simulink model "PowerSplitHEV_system_model"  (R2023a)
settings: Solver=daessc  StartTime=0.0  StopTime=t_end  RelTol=1e-3  AbsTol=1e-3  EnableMultiTasking=on
PreLoadFcn:
  | PowerSplitHEV_params
  | 
  | PowerSplitHEV_DirectInput_selectInput
PostLoadFcn:
  | % Load external input signals
  | % based on the referenced subsystem
  | % for the Controller & Environment block.
  | PowerSplitHEV_system_model_setup
libraries: fl_lib x1, nesl_utility x1
settings Model: Creator=MathWorks  LastModifiedBy=isaacito
settings SolverCC: AutoScaleAbsTol=off  DaesscMode=Fast  AlgebraicLoopSolver=TrustRegion
settings DataIOCC: LimitDataPoints=on  MaxDataPoints=15000  SaveFormat=Array  DSMLogging=off  InspectSignalLogs=on
settings OptimizationCC: ReuseModelBlockBuffer=off  ExpressionDepthLimit=2147483647  LifeSpan=inf
settings DebuggingCC: UnconnectedInputMsg=warning  UnconnectedOutputMsg=warning  UnconnectedLineMsg=warning  StateNameClashWarn=warning  SFUnexpectedBacktrackingDiag=warning  SFNoUnconditionalDefaultTransitionDiag=warning  SFExecutionAtInitializationDiag=none  ArithmeticOperatorsInVariantConditions=warning
settings HardwareCC: ProdBitPerPointer=32  ProdBitPerSizeT=32  ProdBitPerPtrDiffT=32  ProdLargestAtomicFloat=None  ProdIntDivRoundTo=Undefined  ProdEndianess=Unspecified  ProdWordSize=32  ProdHWDeviceType=32-bit Generic
settings ModelReferenceCC: EnableRefExpFcnMdlSchedulingChecks=on  PropagateSignalLabelsOutOfModel=off
settings SFSimCC: SimUseLocalCustomCode=off  CustomCodeUndefinedFunction=UseInterfaceOnly
settings RTWCC: RTWUseLocalCustomCode=off  DLArmComputeVersion=19.05
settings CodeAppCC: StateflowObjectComments=on
settings GRTTargetCC: TargetLangStandard=C89/C90 (ANSI)  CombineOutputUpdateFcns=off  GRTInterface=on
settings ConfigComp: CovMetricSettings=dw  CovSaveCumulativeToWorkspaceVar=on  CovSaveSingleToWorkspaceVar=on  CovExternalEMLEnable=off
settings SimscapeCC: SimscapeLogType=all  SimscapeLogSimulationStatistics=on  SimscapeLogLimitData=off  SimscapeLogDataHistory=10000

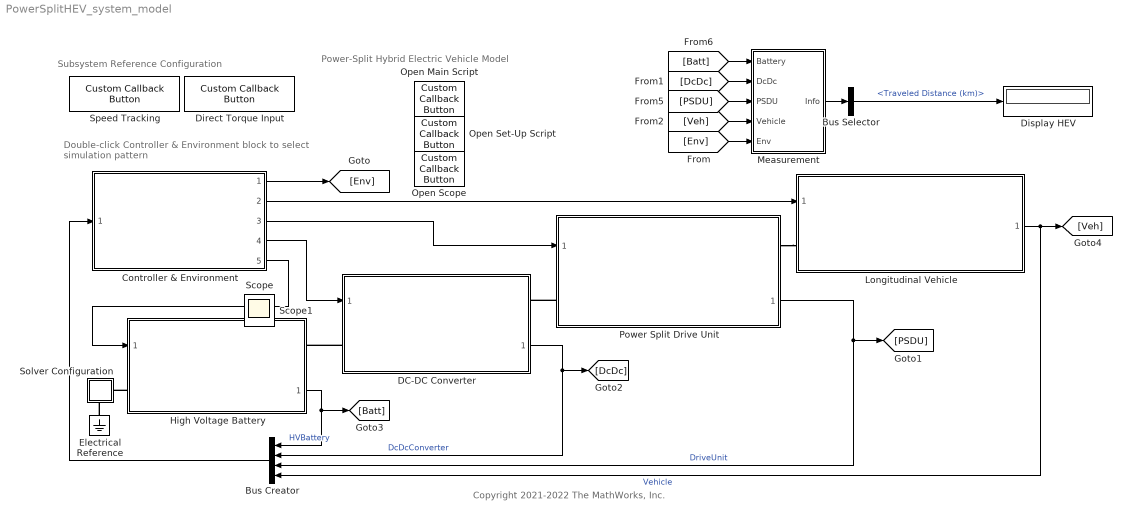
== system PowerSplitHEV_system_model ==
  note: Double-click Controller & Environment block
      | to select simulation pattern
  note: Subsystem Reference Configuration
  note: Power-Split Hybrid Electric Vehicle Model
  note: Copyright 2021-2022 The MathWorks, Inc.
  Bus Creator : BusCreator  Inputs=4
  Bus Selector : BusSelector  OutputSignals=Traveled Distance (km)
  Controller & Environment : Subsystem  ReferencedSubsystem=PowerSplitHEV_SpeedTracking_refsub
  DC-DC Converter : Subsystem  ReferencedSubsystem=DcDcConverterElec_refsub
      settings: PortSchema="{\"entries\":[{\"content\":{\"sides\":[{\"content\":{\"connectorIds\":[\"In1\",\"LConn1\"]},\"type\":\"ConnectorPlacement.EquallySpacedRectSide\",\"uuid\":\"9fe8411b-04be-463e-9924-e5b159c802ea\"},{\"content\":{\"connectorIds\":[\"RConn1\",\"Out1\"],\"side\":\"RIGHT\"},\"type\":\"ConnectorPlacement.EquallySpacedRectSide\",\"uuid\":\"f74ab51b-f871-4eba-ad48-2355a260a50e\"},{\"content\":{\"side\":\"TOP\"},\"type\":\"ConnectorPlacement.EquallySpacedRectSide\",\"uuid\":\"5fe4b190-e251-4a98-9e87-336539b68eba\"},{\"content\":{\"side\":\"HIDDEN\"},\"type\":\"ConnectorPlacement.EquallySpacedRectSide\",\"uuid\":\"70e61028-3020-42d1-b1c6-53691d04cdd7\"}]},\"type\":\"ConnectorPlacement.EquallySpacedConnector\",\"uuid\":\"64b2eeb8-79e5-4be4-98bc-81a0cbd61baa\"}],\"packageUris\":[\"http://schema.mathworks.com/mf0/Connector/R2020b\"],\"version\":\"1.0\"}"
  Direct Torque Input : CustomCallbackButton  Configuration="{\"components\":[{\"name\":\"BackgroundImageComponent\",\"settings\":{\"image\":{\"size\":[0,0],\"src\":\"default\",\"srcOrientation\":\"Right\"},\"position\":[0,0,1,1]}},{\"name\":\"ButtonStateComponent\",\"settings\":{\"buttonType\":\"momentary\",\"clickFcn\":\"disp(\\\"Selecting referenced subsystem: \\\" + ...\\n  \\\"Direct torque input\\\")\\n\\nset_param( gcs + \\\"\\/Controller & Environment\\\", ...\\n  \\\"ReferencedSubsystem\\\", ...\\n  \\\"PowerSplitHEV_DirectInput_refsub\\\");\\n\\nPowerSplitHEV_DirectInput_selectInput( ...\\n  \\\"InputPattern\\\", \\\"PowerSplitDrive\\\", ...\\n  \\\"DisplayMessage\\\", true );\\n\",\"onValue\":1,\"position\":[0,0,1,1],\"pressDelay\":\"500\",\"pressFcn\":\"\",\"repeatInterval\":\"0\",\"states\":[{\"horizontalAlignment\":\"center\",\"image\":{\"position\":[0,0,1,1],\"src\":\"default\",\"srcOrientation\":\"Right\"},\"label\":{\"color\":[0.01176470588,0.01176470588,0.01176470588,1],\"icon\":{\"size\":[0,0],\"src\":\"default\",\"srcOrientation\":\"Right\"},\"iconPlacement\":\"left\",\"text\":{\"content\":\"Select\"}},\"labelOffset\":[0,0],\"verticalAlignment\":\"middle\"},{\"horizontalAlignment\":\"center\",\"image\":{\"position\":[0,0,1,1],\"src\":\"default\",\"srcOrientation\":\"Right\"},\"label\":{\"color\":[0.01176470588,0.01176470588,0.01176470588,1],\"icon\":{\"size\":[0,0],\"src\":\"default\",\"srcOrientation\":\"Right\"},\"iconPlacement\":\"left\",\"text\":{\"content\":\"Select\"}},\"labelOffset\":[0,0],\"verticalAlignment\":\"middle\"},{\"horizontalAlignment\":\"center\",\"image\":{\"position\":[0,0,1,1],\"src\":\"default\",\"srcOrientation\":\"Right\"},\"label\":{\"color\":[0.01176470588,0.01176470588,0.01176470588,1],\"icon\":{\"size\":[0,0],\"src\":\"default\",\"srcOrientation\":\"Right\"},\"iconPlacement\":\"left\",\"text\":{\"content\":\"Select\"}},\"labelOffset\":[0,0],\"verticalAlignment\":\"middle\"},{\"horizontalAlignment\":\"center\",\"image\":{\"position\":[0,0,1,1],\"src\":\"default\",\"srcOrientation\":\"Right\"},\"label\":{\"color\":[0.01176470588,0.01176470588,0.01176470588,1],\"icon\":{\"size\":[0,0],\"src\":\"default\",\"srcOrientation\":\"Right\"},\"iconPlacement\":\"left\",\"text\":{\"content\":\"Select\"}},\"labelOffset\":[0,0],\"verticalAlignment\":\"middle\"}]}},{\"name\":\"ForegroundImageComponent\",\"settings\":{\"image\":{\"size\":[0,0],\"src\":\"default\",\"srcOrientation\":\"Right\"},\"isForeground\":1,\"position\":[0,0,1,1]}}],\"settings\":{\"BindingType\":\"standalone\",\"backgroundColor\":[244,244,244,1],\"backgroundOffset\":0.2,\"backgroundOpacity\":1,\"fixedAspectRatio\":\"off\",\"foregroundColor\":[0.01176470588,0.01176470588,0.01176470588,1],\"migratedFromLegacy\":true,\"useBackgroundColor\":true,\"variant\":\"callback\",\"version\":\"R2023a\"},\"type\":\"Button\"}"  CustomBackgroundColor="{\"color\":[0.9568627451,0.9568627451,0.9568627451],\"show\":true}"
  Display HEV : Display
  Electrical Reference : fl_lib/Electrical/Electrical Elements/Electrical Reference
  High Voltage Battery : Subsystem  ReferencedSubsystem=BatteryHV_refsub_Basic
      settings: OpenFcn="open_system(gcb, \"force\")"  PortSchema="{\"entries\":[{\"content\":{\"sides\":[{\"content\":{\"connectorIds\":[\"In1\",\"LConn1\"]},\"type\":\"ConnectorPlacement.EquallySpacedRectSide\",\"uuid\":\"9fe8411b-04be-463e-9924-e5b159c802ea\"},{\"content\":{\"connectorIds\":[\"RConn1\",\"Out1\"],\"side\":\"RIGHT\"},\"type\":\"ConnectorPlacement.EquallySpacedRectSide\",\"uuid\":\"f74ab51b-f871-4eba-ad48-2355a260a50e\"},{\"content\":{\"side\":\"TOP\"},\"type\":\"ConnectorPlacement.EquallySpacedRectSide\",\"uuid\":\"5fe4b190-e251-4a98-9e87-336539b68eba\"},{\"content\":{\"side\":\"HIDDEN\"},\"type\":\"ConnectorPlacement.EquallySpacedRectSide\",\"uuid\":\"70e61028-3020-42d1-b1c6-53691d04cdd7\"}]},\"type\":\"ConnectorPlacement.EquallySpacedConnector\",\"uuid\":\"64b2eeb8-79e5-4be4-98bc-81a0cbd61baa\"}],\"packageUris\":[\"http://schema.mathworks.com/mf0/Connector/R2020b\"],\"version\":\"1.0\"}"
  Longitudinal Vehicle : Subsystem  ReferencedSubsystem=Vehicle1D_refsub_Basic
  Measurement : Subsystem
  Open Main Script : CustomCallbackButton  Configuration="{\"components\":[{\"name\":\"BackgroundImageComponent\",\"settings\":{\"image\":{\"size\":[0,0],\"src\":\"default\",\"srcOrientation\":\"Right\"},\"position\":[0,0,1,1]}},{\"name\":\"ButtonStateComponent\",\"settings\":{\"buttonType\":\"momentary\",\"clickFcn\":\"edit(\\\"PowerSplitHEV_main_script\\\")\\n\",\"onValue\":1,\"position\":[0,0,1,1],\"pressDelay\":\"500\",\"pressFcn\":\"\",\"repeatInterval\":\"0\",\"states\":[{\"horizontalAlignment\":\"center\",\"image\":{\"position\":[0,0,1,1],\"src\":\"default\",\"srcOrientation\":\"Right\"},\"label\":{\"color\":[0.01176470588,0.01176470588,0.01176470588,1],\"icon\":{\"size\":[0,0],\"src\":\"default\",\"srcOrientation\":\"Right\"},\"iconPlacement\":\"left\",\"text\":{\"content\":\"Open\"}},\"labelOffset\":[0,0],\"verticalAlignment\":\"middle\"},{\"horizontalAlignment\":\"center\",\"image\":{\"position\":[0,0,1,1],\"src\":\"default\",\"srcOrientation\":\"Right\"},\"label\":{\"color\":[0.01176470588,0.01176470588,0.01176470588,1],\"icon\":{\"size\":[0,0],\"src\":\"default\",\"srcOrientation\":\"Right\"},\"iconPlacement\":\"left\",\"text\":{\"content\":\"Open\"}},\"labelOffset\":[0,0],\"verticalAlignment\":\"middle\"},{\"horizontalAlignment\":\"center\",\"image\":{\"position\":[0,0,1,1],\"src\":\"default\",\"srcOrientation\":\"Right\"},\"label\":{\"color\":[0.01176470588,0.01176470588,0.01176470588,1],\"icon\":{\"size\":[0,0],\"src\":\"default\",\"srcOrientation\":\"Right\"},\"iconPlacement\":\"left\",\"text\":{\"content\":\"Open\"}},\"labelOffset\":[0,0],\"verticalAlignment\":\"middle\"},{\"horizontalAlignment\":\"center\",\"image\":{\"position\":[0,0,1,1],\"src\":\"default\",\"srcOrientation\":\"Right\"},\"label\":{\"color\":[0.01176470588,0.01176470588,0.01176470588,1],\"icon\":{\"size\":[0,0],\"src\":\"default\",\"srcOrientation\":\"Right\"},\"iconPlacement\":\"left\",\"text\":{\"content\":\"Open\"}},\"labelOffset\":[0,0],\"verticalAlignment\":\"middle\"}]}},{\"name\":\"ForegroundImageComponent\",\"settings\":{\"image\":{\"size\":[0,0],\"src\":\"default\",\"srcOrientation\":\"Right\"},\"isForeground\":1,\"position\":[0,0,1,1]}}],\"settings\":{\"BindingType\":\"standalone\",\"backgroundColor\":[244,244,244,1],\"backgroundOffset\":0.2,\"backgroundOpacity\":1,\"fixedAspectRatio\":\"off\",\"foregroundColor\":[0.01176470588,0.01176470588,0.01176470588,1],\"migratedFromLegacy\":true,\"useBackgroundColor\":true,\"variant\":\"callback\",\"version\":\"R2023a\"},\"type\":\"Button\"}"  CustomBackgroundColor="{\"color\":[0.9568627451,0.9568627451,0.9568627451],\"show\":true}"
  Open Scope : CustomCallbackButton  Configuration="{\"components\":[{\"name\":\"BackgroundImageComponent\",\"settings\":{\"image\":{\"size\":[0,0],\"src\":\"default\",\"srcOrientation\":\"Right\"},\"position\":[0,0,1,1]}},{\"name\":\"ButtonStateComponent\",\"settings\":{\"buttonType\":\"momentary\",\"clickFcn\":\"open_system(gcs + \\\"\\/Measurement\\/Scope HEV\\\")\",\"onValue\":1,\"position\":[0,0,1,1],\"pressDelay\":\"500\",\"pressFcn\":\"\",\"repeatInterval\":\"0\",\"states\":[{\"horizontalAlignment\":\"center\",\"image\":{\"position\":[0,0,1,1],\"src\":\"default\",\"srcOrientation\":\"Right\"},\"label\":{\"color\":[0.01176470588,0.01176470588,0.01176470588,1],\"icon\":{\"size\":[0,0],\"src\":\"default\",\"srcOrientation\":\"Right\"},\"iconPlacement\":\"left\",\"text\":{\"content\":\"Open\"}},\"labelOffset\":[0,0],\"verticalAlignment\":\"middle\"},{\"horizontalAlignment\":\"center\",\"image\":{\"position\":[0,0,1,1],\"src\":\"default\",\"srcOrientation\":\"Right\"},\"label\":{\"color\":[0.01176470588,0.01176470588,0.01176470588,1],\"icon\":{\"size\":[0,0],\"src\":\"default\",\"srcOrientation\":\"Right\"},\"iconPlacement\":\"left\",\"text\":{\"content\":\"Open\"}},\"labelOffset\":[0,0],\"verticalAlignment\":\"middle\"},{\"horizontalAlignment\":\"center\",\"image\":{\"position\":[0,0,1,1],\"src\":\"default\",\"srcOrientation\":\"Right\"},\"label\":{\"color\":[0.01176470588,0.01176470588,0.01176470588,1],\"icon\":{\"size\":[0,0],\"src\":\"default\",\"srcOrientation\":\"Right\"},\"iconPlacement\":\"left\",\"text\":{\"content\":\"Open\"}},\"labelOffset\":[0,0],\"verticalAlignment\":\"middle\"},{\"horizontalAlignment\":\"center\",\"image\":{\"position\":[0,0,1,1],\"src\":\"default\",\"srcOrientation\":\"Right\"},\"label\":{\"color\":[0.01176470588,0.01176470588,0.01176470588,1],\"icon\":{\"size\":[0,0],\"src\":\"default\",\"srcOrientation\":\"Right\"},\"iconPlacement\":\"left\",\"text\":{\"content\":\"Open\"}},\"labelOffset\":[0,0],\"verticalAlignment\":\"middle\"}]}},{\"name\":\"ForegroundImageComponent\",\"settings\":{\"image\":{\"size\":[0,0],\"src\":\"default\",\"srcOrientation\":\"Right\"},\"isForeground\":1,\"position\":[0,0,1,1]}}],\"settings\":{\"BindingType\":\"standalone\",\"backgroundColor\":[244,244,244,1],\"backgroundOffset\":0.2,\"backgroundOpacity\":1,\"fixedAspectRatio\":\"off\",\"foregroundColor\":[0.01176470588,0.01176470588,0.01176470588,1],\"migratedFromLegacy\":true,\"useBackgroundColor\":true,\"variant\":\"callback\",\"version\":\"R2023a\"},\"type\":\"Button\"}"  CustomBackgroundColor="{\"color\":[0.9568627451,0.9568627451,0.9568627451],\"show\":true}"
  Open Set-Up Script : CustomCallbackButton  Configuration="{\"components\":[{\"name\":\"BackgroundImageComponent\",\"settings\":{\"image\":{\"size\":[0,0],\"src\":\"default\",\"srcOrientation\":\"Right\"},\"position\":[0,0,1,1]}},{\"name\":\"ButtonStateComponent\",\"settings\":{\"buttonType\":\"momentary\",\"clickFcn\":\"edit(\\\"PowerSplitHEV_params\\\")\\n\",\"onValue\":1,\"position\":[0,0,1,1],\"pressDelay\":\"500\",\"pressFcn\":\"\",\"repeatInterval\":\"0\",\"states\":[{\"horizontalAlignment\":\"center\",\"image\":{\"position\":[0,0,1,1],\"src\":\"default\",\"srcOrientation\":\"Right\"},\"label\":{\"color\":[0.01176470588,0.01176470588,0.01176470588,1],\"icon\":{\"size\":[0,0],\"src\":\"default\",\"srcOrientation\":\"Right\"},\"iconPlacement\":\"left\",\"text\":{\"content\":\"Open\"}},\"labelOffset\":[0,0],\"verticalAlignment\":\"middle\"},{\"horizontalAlignment\":\"center\",\"image\":{\"position\":[0,0,1,1],\"src\":\"default\",\"srcOrientation\":\"Right\"},\"label\":{\"color\":[0.01176470588,0.01176470588,0.01176470588,1],\"icon\":{\"size\":[0,0],\"src\":\"default\",\"srcOrientation\":\"Right\"},\"iconPlacement\":\"left\",\"text\":{\"content\":\"Open\"}},\"labelOffset\":[0,0],\"verticalAlignment\":\"middle\"},{\"horizontalAlignment\":\"center\",\"image\":{\"position\":[0,0,1,1],\"src\":\"default\",\"srcOrientation\":\"Right\"},\"label\":{\"color\":[0.01176470588,0.01176470588,0.01176470588,1],\"icon\":{\"size\":[0,0],\"src\":\"default\",\"srcOrientation\":\"Right\"},\"iconPlacement\":\"left\",\"text\":{\"content\":\"Open\"}},\"labelOffset\":[0,0],\"verticalAlignment\":\"middle\"},{\"horizontalAlignment\":\"center\",\"image\":{\"position\":[0,0,1,1],\"src\":\"default\",\"srcOrientation\":\"Right\"},\"label\":{\"color\":[0.01176470588,0.01176470588,0.01176470588,1],\"icon\":{\"size\":[0,0],\"src\":\"default\",\"srcOrientation\":\"Right\"},\"iconPlacement\":\"left\",\"text\":{\"content\":\"Open\"}},\"labelOffset\":[0,0],\"verticalAlignment\":\"middle\"}]}},{\"name\":\"ForegroundImageComponent\",\"settings\":{\"image\":{\"size\":[0,0],\"src\":\"default\",\"srcOrientation\":\"Right\"},\"isForeground\":1,\"position\":[0,0,1,1]}}],\"settings\":{\"BindingType\":\"standalone\",\"backgroundColor\":[244,244,244,1],\"backgroundOffset\":0.2,\"backgroundOpacity\":1,\"fixedAspectRatio\":\"off\",\"foregroundColor\":[0.01176470588,0.01176470588,0.01176470588,1],\"migratedFromLegacy\":true,\"useBackgroundColor\":true,\"variant\":\"callback\",\"version\":\"R2023a\"},\"type\":\"Button\"}"  CustomBackgroundColor="{\"color\":[0.9568627451,0.9568627451,0.9568627451],\"show\":true}"
  Power Split Drive Unit : Subsystem  ReferencedSubsystem=PowerSplitDriveUnit_refsub_Basic
      settings: PortSchema="{\"entries\":[{\"content\":{\"sides\":[{\"content\":{\"connectorIds\":[\"In1\",\"LConn1\"]},\"type\":\"ConnectorPlacement.EquallySpacedRectSide\",\"uuid\":\"974aedaf-bb26-4d59-a293-409346043c39\"},{\"content\":{\"connectorIds\":[\"RConn1\",\"Out1\"],\"side\":\"RIGHT\"},\"type\":\"ConnectorPlacement.EquallySpacedRectSide\",\"uuid\":\"12ed2c12-3442-42d2-9925-d6af8f0a29b3\"},{\"content\":{\"side\":\"TOP\"},\"type\":\"ConnectorPlacement.EquallySpacedRectSide\",\"uuid\":\"599325fb-3fa7-4117-9978-1ddfbbeb0247\"},{\"content\":{\"side\":\"HIDDEN\"},\"type\":\"ConnectorPlacement.EquallySpacedRectSide\",\"uuid\":\"40453f65-ace7-4c7b-ae3d-0c837e197c38\"}]},\"type\":\"ConnectorPlacement.EquallySpacedConnector\",\"uuid\":\"841da484-ce2c-414e-826b-1cb66c55f7d7\"}],\"packageUris\":[\"http://schema.mathworks.com/mf0/Connector/R2020b\"],\"version\":\"1.0\"}"
  Solver Configuration : Subsystem
      settings: PortSchema="{\"entries\":[{\"content\":{\"sides\":[{\"content\":{\"connectorIds\":[]},\"type\":\"ConnectorPlacement.EquallySpacedRectSide\",\"uuid\":\"4a7e26c2-e9e9-4fea-b605-533b1a682be7\"},{\"content\":{\"connectorIds\":[\"RConn1\"],\"side\":\"RIGHT\"},\"type\":\"ConnectorPlacement.EquallySpacedRectSide\",\"uuid\":\"0210e324-555e-4372-b836-fcc8ab23e933\"},{\"content\":{\"connectorIds\":[],\"side\":\"TOP\"},\"type\":\"ConnectorPlacement.EquallySpacedRectSide\",\"uuid\":\"9bbae011-e6fc-4534-a44f-d79a5697c939\"},{\"content\":{\"connectorIds\":[\"RConn2\"],\"side\":\"BOTTOM\"},\"type\":\"ConnectorPlacement.EquallySpacedRectSide\",\"uuid\":\"d5829c0a-26ea-402d-a1c6-900997ddf1a8\"}]},\"type\":\"ConnectorPlacement.EquallySpacedConnector\",\"uuid\":\"f4e17c65-54c6-42fe-a467-9c6b014b697a\"}],\"packageUris\":[\"http://schema.mathworks.com/mf0/Connector/19700101\"],\"version\":\"1.0\"}"
  Speed Tracking : CustomCallbackButton  Configuration="{\"components\":[{\"name\":\"BackgroundImageComponent\",\"settings\":{\"image\":{\"size\":[0,0],\"src\":\"default\",\"srcOrientation\":\"Right\"},\"position\":[0,0,1,1]}},{\"name\":\"ButtonStateComponent\",\"settings\":{\"buttonType\":\"momentary\",\"clickFcn\":\"disp(\\\"Selecting referenced subsystem: \\\" + ...\\n  \\\"Speed tracking\\\")\\n\\nset_param( gcs + \\\"\\/Controller & Environment\\\", ...\\n  \\\"ReferencedSubsystem\\\", ...\\n  \\\"PowerSplitHEV_SpeedTracking_refsub\\\");\\n\\nPowerSplitHEV_SpeedTracking_selectInput( ...\\n  \\\"InputPattern\\\", \\\"SimpleDrivePattern\\\", ...\\n  \\\"DisplayMessage\\\", true );\\n\",\"onValue\":1,\"position\":[0,0,1,1],\"pressDelay\":\"500\",\"pressFcn\":\"\",\"repeatInterval\":\"0\",\"states\":[{\"horizontalAlignment\":\"center\",\"image\":{\"position\":[0,0,1,1],\"src\":\"default\",\"srcOrientation\":\"Right\"},\"label\":{\"color\":[0.01176470588,0.01176470588,0.01176470588,1],\"icon\":{\"size\":[0,0],\"src\":\"default\",\"srcOrientation\":\"Right\"},\"iconPlacement\":\"left\",\"text\":{\"content\":\"Select\"}},\"labelOffset\":[0,0],\"verticalAlignment\":\"middle\"},{\"horizontalAlignment\":\"center\",\"image\":{\"position\":[0,0,1,1],\"src\":\"default\",\"srcOrientation\":\"Right\"},\"label\":{\"color\":[0.01176470588,0.01176470588,0.01176470588,1],\"icon\":{\"size\":[0,0],\"src\":\"default\",\"srcOrientation\":\"Right\"},\"iconPlacement\":\"left\",\"text\":{\"content\":\"Select\"}},\"labelOffset\":[0,0],\"verticalAlignment\":\"middle\"},{\"horizontalAlignment\":\"center\",\"image\":{\"position\":[0,0,1,1],\"src\":\"default\",\"srcOrientation\":\"Right\"},\"label\":{\"color\":[0.01176470588,0.01176470588,0.01176470588,1],\"icon\":{\"size\":[0,0],\"src\":\"default\",\"srcOrientation\":\"Right\"},\"iconPlacement\":\"left\",\"text\":{\"content\":\"Select\"}},\"labelOffset\":[0,0],\"verticalAlignment\":\"middle\"},{\"horizontalAlignment\":\"center\",\"image\":{\"position\":[0,0,1,1],\"src\":\"default\",\"srcOrientation\":\"Right\"},\"label\":{\"color\":[0.01176470588,0.01176470588,0.01176470588,1],\"icon\":{\"size\":[0,0],\"src\":\"default\",\"srcOrientation\":\"Right\"},\"iconPlacement\":\"left\",\"text\":{\"content\":\"Select\"}},\"labelOffset\":[0,0],\"verticalAlignment\":\"middle\"}]}},{\"name\":\"ForegroundImageComponent\",\"settings\":{\"image\":{\"size\":[0,0],\"src\":\"default\",\"srcOrientation\":\"Right\"},\"isForeground\":1,\"position\":[0,0,1,1]}}],\"settings\":{\"BindingType\":\"standalone\",\"backgroundColor\":[244,244,244,1],\"backgroundOffset\":0.2,\"backgroundOpacity\":1,\"fixedAspectRatio\":\"off\",\"foregroundColor\":[0.01176470588,0.01176470588,0.01176470588,1],\"migratedFromLegacy\":true,\"useBackgroundColor\":true,\"variant\":\"callback\",\"version\":\"R2023a\"},\"type\":\"Button\"}"  CustomBackgroundColor="{\"color\":[0.9568627451,0.9568627451,0.9568627451],\"show\":true}"
  Scope : Scope
  Scope1 : Scope
  wires:
  Longitudinal Vehicle/1 -> [Veh], Bus Creator/4  "Vehicle"
  Measurement/1(Info) -> Bus Selector/1
  High Voltage Battery/1 -> Bus Creator/1, [Batt]  "HVBattery"
  Bus Selector/1 -> Display HEV/1  "<Traveled Distance (km)>"
  Power Split Drive Unit/1 -> Bus Creator/3, [PSDU]  "DriveUnit"
  Controller & Environment/1 -> [Env]
  Bus Creator/1 -> Controller & Environment/1
  DC-DC Converter/1 -> Bus Creator/2, [DcDc]  "DcDcConverter"
  Controller & Environment/4 -> DC-DC Converter/1
  Controller & Environment/5 -> High Voltage Battery/1
  [DcDc] -> Measurement/2(DcDc)
  [Veh] -> Measurement/4(Vehicle)
  [Batt] -> Measurement/1(Battery)
  [PSDU] -> Measurement/3(PSDU)
  [Env] -> Measurement/5(Env)
  Controller & Environment/2 -> Longitudinal Vehicle/1
  Controller & Environment/3 -> Power Split Drive Unit/1
  connections:
  High Voltage Battery/LConn1 -- Solver Configuration/RConn1
  Electrical Reference/LConn1 -- Solver Configuration/RConn2
  DC-DC Converter/LConn1 -- High Voltage Battery/RConn1
  Power Split Drive Unit/LConn1 -- DC-DC Converter/RConn1
  Power Split Drive Unit/RConn1 -- Longitudinal Vehicle/LConn1

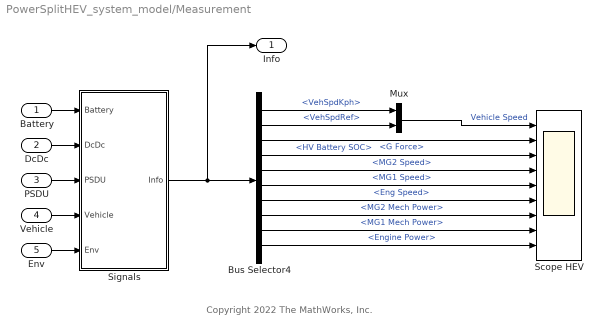
== system PowerSplitHEV_system_model/Measurement ==
  note: Copyright 2022 The MathWorks, Inc.
  Battery : Inport
  DcDc : Inport  Port=2
  PSDU : Inport  Port=3
  Vehicle : Inport  Port=4
  Env : Inport  Port=5
  Bus Selector4 : BusSelector  OutputSignals=VehSpdKph,VehSpdRef,G Force,HV Battery SOC,MG2 Speed,MG1 Speed,Eng Speed,MG2 Mech Power,MG1 Mech Power,Engine Power
  Mux : Mux  Inputs=2
  Scope HEV : Scope  NumInputPorts=9
  Signals : Subsystem
  Info : Outport
  wires:
  Bus Selector4/7 -> Scope HEV/6  "<Eng Speed>"
  Bus Selector4/10 -> Scope HEV/9  "<Engine Power>"
  Bus Selector4/5 -> Scope HEV/4  "<MG2 Speed>"
  Bus Selector4/3 -> Scope HEV/2  "<G Force>"
  Bus Selector4/9 -> Scope HEV/8  "<MG1 Mech Power>"
  Bus Selector4/8 -> Scope HEV/7  "<MG2 Mech Power>"
  Mux/1 -> Scope HEV/1  "Vehicle Speed"
  Bus Selector4/4 -> Scope HEV/3  "<HV Battery SOC>"
  Bus Selector4/1 -> Mux/1  "<VehSpdKph>"
  Bus Selector4/2 -> Mux/2  "<VehSpdRef>"
  Bus Selector4/6 -> Scope HEV/5  "<MG1 Speed>"
  Signals/1(Info) -> Info/1, Bus Selector4/1
  Battery/1 -> Signals/1(Battery)
  DcDc/1 -> Signals/2(DcDc)
  PSDU/1 -> Signals/3(PSDU)
  Vehicle/1 -> Signals/4(Vehicle)
  Env/1 -> Signals/5(Env)

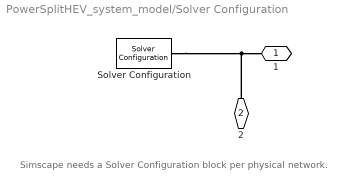
== system PowerSplitHEV_system_model/Solver Configuration ==
  note: Simscape needs a Solver Configuration block per physical network.
  Solver Configuration : nesl_utility/Solver Configuration  PhysicalDomain=network_engine_domain  SubClassName=solver  LeftPortType=input  RightPortType=generic  Tones=[]  Harmonics=[]  SimulateNoise=off  Profile=off  UseLocalSampling=off  EnableSwitchedLinearOptims=on  FrequencyDomain=off  UseCCode=off  RelTol=0.001  AbsTol=1e-06  MinStep=1e-09  ToWorkspace=off  RevertToSquareIcSolve=off  NumHomotopyIterations=100  PhasorMode=off  PhasorModeNumHarmonics=1  ConsistencySolver=NEWTON_FTOL  IndexReductionMethod=DerivativeReplacement  DoDC=off  ResidualTolerance=1e-9  ConsistencyTolSource=GLOBAL  ConsistencyAbsTol=0.001  ConsistencyRelTol=0.001  ConsistencyTolFactor=0.001  UseLocalSolver=off  LocalSolverChoice=NE_BACKWARD_EULER_ADVANCER  ResolveIndetEquations=on  FunctionEvalNumThread=1  LocalSolverSampleTime=0.01  DoFixedCost=off  MaxNonlinIter=3  MaxModeIter=2  ComputeImpulses=off  ImpulseIterations=2  LinearAlgebra=auto  LinearAlgebraNumThread=0  EquationFormulation=NE_TIME_EF  DelaysMemoryBudget=1024  AutomaticFiltering=on  FilteringTimeConstant=0.001  PartitionStorageMethod=AS_NEEDED  PartitionMemoryBudget=1024  PartitionMethod=FAST
      settings: AttributesFormatString=Local solver %<UseLocalSolver>
  1 : PMIOPort  Side=Right
  2 : PMIOPort  Port=2  Side=Right
  connections:
  Solver Configuration/RConn1 -- 1/RConn1 -- 2/RConn1

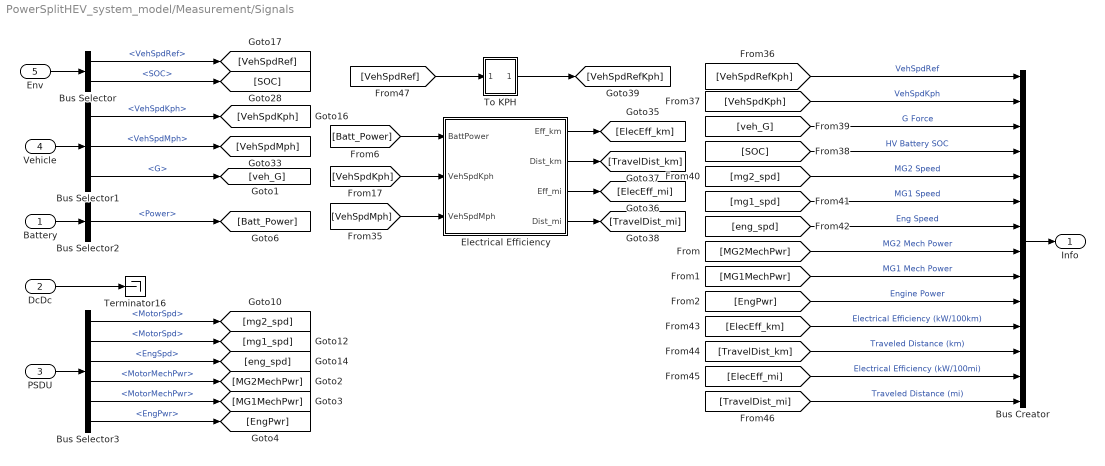
== system PowerSplitHEV_system_model/Measurement/Signals ==
  Battery : Inport
  DcDc : Inport  Port=2
  PSDU : Inport  Port=3
  Vehicle : Inport  Port=4
  Env : Inport  Port=5
  Bus Creator : BusCreator  Inputs=14
  Bus Selector : BusSelector  OutputSignals=VehSpdRef,SOC
  Bus Selector1 : BusSelector  OutputSignals=VehSpdKph,VehSpdMph,G
  Bus Selector2 : BusSelector  OutputSignals=Power
  Bus Selector3 : BusSelector  OutputSignals=mg2.MotorSpd,mg1.MotorSpd,eng.EngSpd,mg2.MotorMechPwr,mg1.MotorMechPwr,eng.EngPwr
  Electrical Efficiency : Subsystem
  Terminator16 : Terminator
  To KPH : Subsystem
  Info : Outport
  wires:
  Bus Selector3/5 -> [MG1MechPwr]  "<MotorMechPwr>"
  [MG2MechPwr] -> Bus Creator/8  "MG2 Mech Power"
  Electrical Efficiency/4(Dist_mi) -> [TravelDist_mi]
  [TravelDist_km] -> Bus Creator/12  "Traveled Distance (km)"
  [EngPwr] -> Bus Creator/10  "Engine Power"
  [VehSpdKph] -> Bus Creator/2  "VehSpdKph"
  [mg2_spd] -> Bus Creator/5  "MG2 Speed"
  [mg1_spd] -> Bus Creator/6  "MG1 Speed"
  [VehSpdMph] -> Electrical Efficiency/3(VehSpdMph)
  [veh_G] -> Bus Creator/3  "G Force"
  [TravelDist_mi] -> Bus Creator/14  "Traveled Distance (mi)"
  Electrical Efficiency/2(Dist_km) -> [TravelDist_km]
  Bus Selector3/6 -> [EngPwr]  "<EngPwr>"
  Bus Selector3/3 -> [eng_spd]  "<EngSpd>"
  Bus Selector/2 -> [SOC]  "<SOC>"
  Bus Selector3/4 -> [MG2MechPwr]  "<MotorMechPwr>"
  Electrical Efficiency/3(Eff_mi) -> [ElecEff_mi]
  [SOC] -> Bus Creator/4  "HV Battery SOC"
  [VehSpdRef] -> To KPH/1(SpdIn)
  [VehSpdKph] -> Electrical Efficiency/2(VehSpdKph)
  [ElecEff_mi] -> Bus Creator/13  "Electrical Efficiency (kW/100mi)"
  [MG1MechPwr] -> Bus Creator/9  "MG1 Mech Power"
  To KPH/1(SpdOut) -> [VehSpdRefKph]
  [VehSpdRefKph] -> Bus Creator/1  "VehSpdRef"
  [Batt_Power] -> Electrical Efficiency/1(BattPower)
  Bus Selector1/2 -> [VehSpdMph]  "<VehSpdMph>"
  [ElecEff_km] -> Bus Creator/11  "Electrical Efficiency (kW/100km)"
  Bus Selector3/2 -> [mg1_spd]  "<MotorSpd>"
  Bus Creator/1 -> Info/1
  Bus Selector1/3 -> [veh_G]  "<G>"
  [eng_spd] -> Bus Creator/7  "Eng Speed"
  Bus Selector1/1 -> [VehSpdKph]  "<VehSpdKph>"
  Electrical Efficiency/1(Eff_km) -> [ElecEff_km]
  Bus Selector2/1 -> [Batt_Power]  "<Power>"
  Bus Selector3/1 -> [mg2_spd]  "<MotorSpd>"
  Bus Selector/1 -> [VehSpdRef]  "<VehSpdRef>"
  DcDc/1 -> Terminator16/1
  Battery/1 -> Bus Selector2/1
  PSDU/1 -> Bus Selector3/1
  Env/1 -> Bus Selector/1
  Vehicle/1 -> Bus Selector1/1

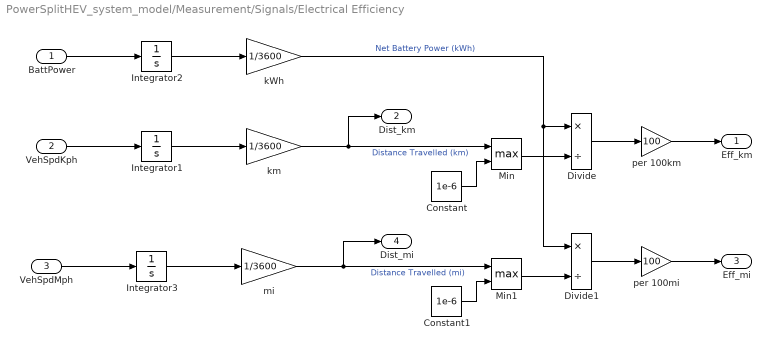
== system PowerSplitHEV_system_model/Measurement/Signals/Electrical Efficiency ==
  BattPower : Inport  Unit=kW
      settings: AttributesFormatString=%<Unit>
  VehSpdKph : Inport  Port=2  Unit=km/hr
      settings: AttributesFormatString=%<Unit>
  VehSpdMph : Inport  Port=3  Unit=mph
      settings: AttributesFormatString=%<Unit>
  Constant : Constant  Value=1e-6
  Constant1 : Constant  Value=1e-6
  Divide : Product  Inputs=*/
  Divide1 : Product  Inputs=*/
  Integrator1 : Integrator
      settings: AttributesFormatString=Initial Condition: %<InitialCondition>
  Integrator2 : Integrator
      settings: AttributesFormatString=Initial Condition: %<InitialCondition>
  Integrator3 : Integrator
      settings: AttributesFormatString=Initial Condition: %<InitialCondition>
  Min : MinMax  Function=max  Inputs=2
  Min1 : MinMax  Function=max  Inputs=2
  kWh : Gain  Gain=1/3600
  km : Gain  Gain=1/3600
  mi : Gain  Gain=1/3600
  per 100km : Gain  Gain=100
  per 100mi : Gain  Gain=100
  Eff_km : Outport
      settings: AttributesFormatString=%<Unit>
  Dist_km : Outport  Port=2  Unit=km
  Eff_mi : Outport  Port=3
      settings: AttributesFormatString=%<Unit>
  Dist_mi : Outport  Port=4  Unit=mi
  wires:
  per 100km/1 -> Eff_km/1
  Min/1 -> Divide/2
  Integrator1/1 -> km/1
  km/1 -> Dist_km/1, Min/1  "Distance Travelled (km)"
  Divide/1 -> per 100km/1
  Constant/1 -> Min/2
  kWh/1 -> Divide1/1, Divide/1  "Net Battery Power (kWh)"
  Integrator2/1 -> kWh/1
  BattPower/1 -> Integrator2/1
  VehSpdKph/1 -> Integrator1/1
  VehSpdMph/1 -> Integrator3/1
  Integrator3/1 -> mi/1
  per 100mi/1 -> Eff_mi/1
  Divide1/1 -> per 100mi/1
  Min1/1 -> Divide1/2
  mi/1 -> Dist_mi/1, Min1/1  "Distance Travelled (mi)"
  Constant1/1 -> Min1/2

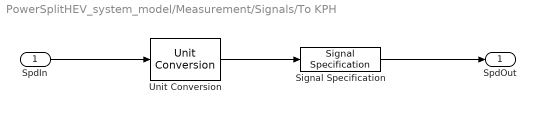
== system PowerSplitHEV_system_model/Measurement/Signals/To KPH ==
  SpdIn : Inport  Unit=m/s
      settings: AttributesFormatString=%<Unit>
  Signal Specification : SignalSpecification  Unit=km/hr
  Unit Conversion : UnitConversion
  SpdOut : Outport  Unit=km/hr
  wires:
  Unit Conversion/1 -> Signal Specification/1
  Signal Specification/1 -> SpdOut/1
  SpdIn/1 -> Unit Conversion/1
